simulink model "radio_FM_simulink_2"  (R2024b)
settings: Solver=FixedStepDiscrete  StartTime=0.0  StopTime=5  FixedStep=sampling_time  RelTol=1e-3
values from neighbouring files (symbols this model uses):
  df = beta*W    (= 450)    [parametros.m]
  epsilon = 1e-8    (= 1e-08)    [parametros.m]
  fc1 = 100.0e3    (= 100000)    [parametros.m]
  fc2 = 98.0e3    (= 98000)    [parametros.m]
  fc3 = 102.0e3    (= 102000)    [parametros.m]
  flo = fc + fi    (= 117000)    [parametros.m]
  sampling_time = 2e-6    (= 2e-06)    [parametros.m]
undefined symbols (not defined in the file or in its folder): dfilt, DiscIntNeverNeededParam
libraries: dsparch4 x2, simulink x1, dspfdesign x1
settings Model: Creator=henao  LastModifiedBy=henao

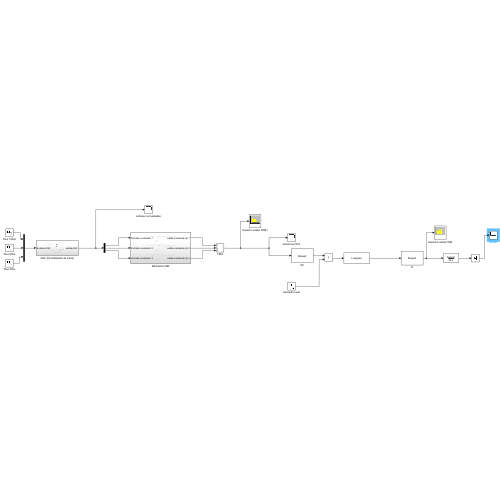
[thumbnail: Simulink's stored preview of the top-level diagram]
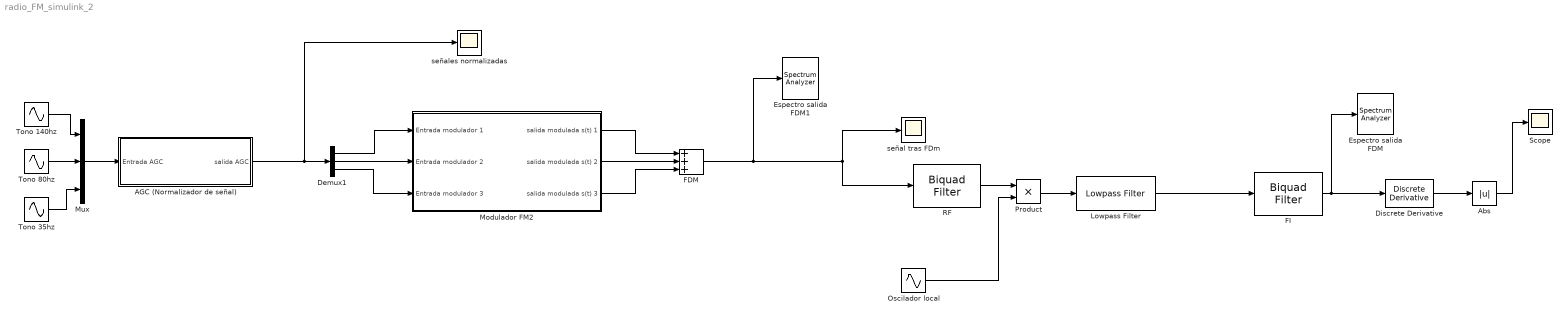
== system radio_FM_simulink_2 ==
  AGC (Normalizador de señal) : Subsystem
  Abs : Abs  SaturateOnIntegerOverflow=off
  Demux1 : Demux  Outputs=3
  Discrete Derivative : simulink/Discrete/Discrete Derivative  gainval=sampling_time  ICPrevScaledInput=0.0  OutMin=[]  OutMax=[]  OutDataType=fixdt(1, 16)  OutScaling=2^-10  DoSatur=off
  Espectro salida FDM : SpectrumAnalyzer  WindowPosition=[93.000000,133.000000,800.000000,500.000000,]  Visible=on  ScopeFrameLocation=window  Method=Welch  PlotAsTwoSidedSpectrum=off  FrequencySpan=Start and stop frequencies  StartFrequency=0  StopFrequency=22000  AveragingMethod=Exponential  YLimits=[-142.21525318,30.44400853]  SelectedToolstripTab=spectrumAnalyzerToolstrip.estimationTab
  Espectro salida FDM1 : SpectrumAnalyzer  WindowPosition=[-48.000000,-225.000000,1440.000000,829.000000,]  Visible=on  ScopeFrameLocation=window  Method=Welch  PlotAsTwoSidedSpectrum=off  FrequencySpan=Start and stop frequencies  StartFrequency=90000  StopFrequency=110000  AveragingMethod=Exponential  YLimits=[-161.96181143721742,129.68025167278262]  SelectedToolstripTab=spectrumAnalyzerToolstrip.channelMeasurementsTab
  FDM : Sum  Inputs=+++
  FI : dsparch4/Biquad Filter  FilterSource=Dialog parameters  CoeffSource=Specify via dialog  FilterObject=dfilt.df2tsos([1 0.3 0.4],[1 0.1 0.2])  IIRFiltStruct=Direct form II transposed  BiQuadCoeffs=sos_fi  ScaleValues=1  IC=0  ICnum=0  ICden=0  a0Flag=Warning  optimizeScaleValues=on  ScaleValueMode=Specify via input port (g)  roundingMode=Floor  overflowMode=off  scaleValueFracLength=14  denProdOutputFracLength=30  denAccumFracLength=30  secondMemoryFracLength=15
      settings: LibrarySourceBlock=dsphdlsupportfiltering/Biquad Filter
  Lowpass Filter : dspfdesign/Lowpass Filter  FilterType=FIR  DesignForMinimumOrder=on  FilterOrder=50  PassbandFrequency=22e3  StopbandFrequency=40e3  PassbandRipple=0.1  StopbandAttenuation=60  SampleRateMode=Specify on dialog  SampleRate=sampling_frec  SimulateUsing=Interpreted execution  roundingMode=Floor  coeffsDataTypeStr=fixdt(1,16)
  Modulador FM2 : Subsystem
  Mux : Mux  Inputs=3
  Oscilador local : Sin  Frequency=2*pi*flo  SampleTime=sampling_time
  Product : Product
  RF : dsparch4/Biquad Filter  FilterSource=Dialog parameters  CoeffSource=Specify via dialog  FilterObject=dfilt.df2tsos([1 0.3 0.4],[1 0.1 0.2])  IIRFiltStruct=Direct form II transposed  BiQuadCoeffs=sos_rf  ScaleValues=1  IC=0  ICnum=0  ICden=0  a0Flag=Warning  optimizeScaleValues=on  ScaleValueMode=Specify via input port (g)  roundingMode=Floor  overflowMode=off  scaleValueFracLength=14  denProdOutputFracLength=30  denAccumFracLength=30  secondMemoryFracLength=15
      settings: LibrarySourceBlock=dsphdlsupportfiltering/Biquad Filter
  Scope : Scope
  Tono 140hz : Sin  Frequency=140*2*pi  SampleTime=sampling_time
  Tono 35hz : Sin  Frequency=35*2*pi  SampleTime=sampling_time
  Tono 80hz : Sin  Frequency=80*2*pi  SampleTime=sampling_time
  señal tras FDm : Scope
  señales normalizadas : Scope
  wires:
  Modulador FM2/2(salida modulada s(t) 2) -> FDM/2
  Modulador FM2/1(salida modulada s(t) 1) -> FDM/1
  Modulador FM2/3(salida modulada s(t) 3) -> FDM/3
  RF/1 -> Product/1
  Oscilador local/1 -> Product/2
  FDM/1 -> Espectro salida FDM1/1, señal tras FDm/1, RF/1
  FI/1 -> Discrete Derivative/1, Espectro salida FDM/1
  Discrete Derivative/1 -> Abs/1
  Abs/1 -> Scope/1
  Lowpass Filter/1 -> FI/1
  Product/1 -> Lowpass Filter/1
  Tono 80hz/1 -> Mux/2
  Tono 35hz/1 -> Mux/3
  Mux/1 -> AGC (Normalizador de señal)/1(Entrada AGC)
  Tono 140hz/1 -> Mux/1
  AGC (Normalizador de señal)/1(salida AGC) -> señales normalizadas/1, Demux1/1
  Demux1/1 -> Modulador FM2/1(Entrada modulador 1)
  Demux1/2 -> Modulador FM2/2(Entrada modulador 2)
  Demux1/3 -> Modulador FM2/3(Entrada modulador 3)

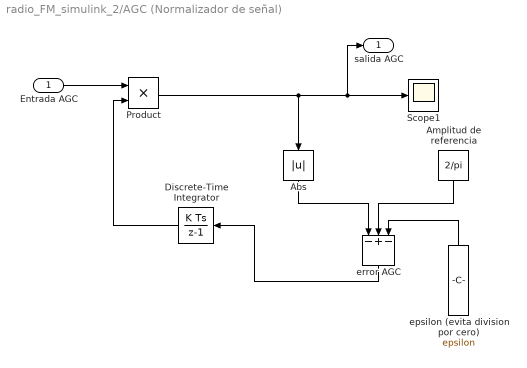
== system radio_FM_simulink_2/AGC (Normalizador de señal) ==
  Entrada AGC : Inport
  Abs : Abs  SaturateOnIntegerOverflow=off
  Amplitud de referencia : Constant  Value=2/pi
  Discrete-Time Integrator : DiscreteIntegrator  gainval=10  SampleTime=sampling_time  ICPrevOutput=DiscIntNeverNeededParam  ICPrevScaledInput=DiscIntNeverNeededParam
  Product : Product
  Scope1 : Scope
  epsilon (evita division por cero) : Constant  Value=epsilon
  error AGC : Sum  Inputs=-+-
  salida AGC : Outport
  wires:
  error AGC/1 -> Discrete-Time Integrator/1
  Product/1 -> Abs/1, salida AGC/1, Scope1/1
  Abs/1 -> error AGC/1
  Amplitud de referencia/1 -> error AGC/2
  epsilon (evita division por cero)/1 -> error AGC/3
  Discrete-Time Integrator/1 -> Product/2
  Entrada AGC/1 -> Product/1

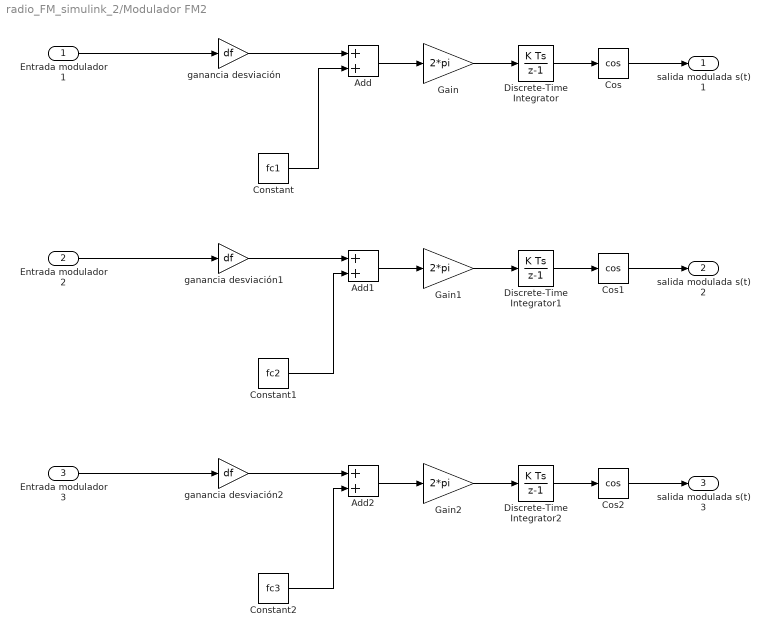
== system radio_FM_simulink_2/Modulador FM2 ==
  Entrada modulador 1 : Inport
  Entrada modulador 2 : Inport  Port=2
  Entrada modulador 3 : Inport  Port=3
  Add : Sum
  Add1 : Sum
  Add2 : Sum
  Constant : Constant  Value=fc1  SampleTime=sampling_time
  Constant1 : Constant  Value=fc2  SampleTime=sampling_time
  Constant2 : Constant  Value=fc3  SampleTime=sampling_time
  Cos : Trigonometry  Operator=cos
  Cos1 : Trigonometry  Operator=cos
  Cos2 : Trigonometry  Operator=cos
  Discrete-Time Integrator : DiscreteIntegrator  gainval=1  SampleTime=sampling_time  ICPrevOutput=DiscIntNeverNeededParam  ICPrevScaledInput=DiscIntNeverNeededParam
  Discrete-Time Integrator1 : DiscreteIntegrator  gainval=1  SampleTime=sampling_time  ICPrevOutput=DiscIntNeverNeededParam  ICPrevScaledInput=DiscIntNeverNeededParam
  Discrete-Time Integrator2 : DiscreteIntegrator  gainval=1  SampleTime=sampling_time  ICPrevOutput=DiscIntNeverNeededParam  ICPrevScaledInput=DiscIntNeverNeededParam
  Gain : Gain  Gain=2*pi
  Gain1 : Gain  Gain=2*pi
  Gain2 : Gain  Gain=2*pi
  ganancia desviación : Gain  Gain=df
  ganancia desviación1 : Gain  Gain=df
  ganancia desviación2 : Gain  Gain=df
  salida modulada s(t) 1 : Outport
  salida modulada s(t) 2 : Outport  Port=2
  salida modulada s(t) 3 : Outport  Port=3
  wires:
  Discrete-Time Integrator/1 -> Cos/1
  Entrada modulador 1/1 -> ganancia desviación/1
  Cos/1 -> salida modulada s(t) 1/1
  Constant/1 -> Add/2
  Add/1 -> Gain/1
  ganancia desviación/1 -> Add/1
  Gain/1 -> Discrete-Time Integrator/1
  Cos1/1 -> salida modulada s(t) 2/1
  ganancia desviación1/1 -> Add1/1
  Constant1/1 -> Add1/2
  Discrete-Time Integrator1/1 -> Cos1/1
  Gain1/1 -> Discrete-Time Integrator1/1
  Add1/1 -> Gain1/1
  Entrada modulador 2/1 -> ganancia desviación1/1
  Add2/1 -> Gain2/1
  Discrete-Time Integrator2/1 -> Cos2/1
  ganancia desviación2/1 -> Add2/1
  Gain2/1 -> Discrete-Time Integrator2/1
  Entrada modulador 3/1 -> ganancia desviación2/1
  Constant2/1 -> Add2/2
  Cos2/1 -> salida modulada s(t) 3/1
